simulink subsystem "Pid_Controller"  (R2025b)
settings: Solver=VariableStepAuto
undefined symbols (not defined in the file): bigBenUpright, pidGains
settings Model: Creator=ahmed medhat  LastModifiedBy=ahmed medhat

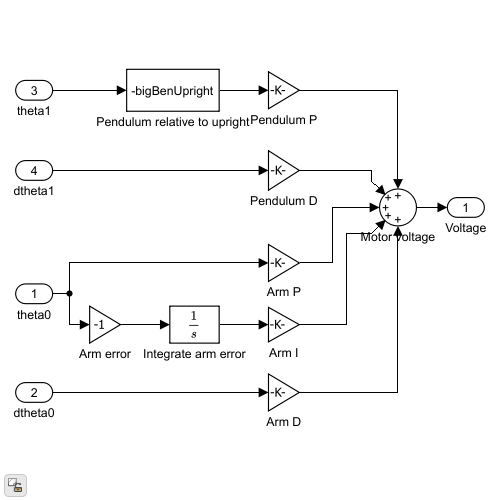
[thumbnail: Simulink's stored preview of the top-level diagram]
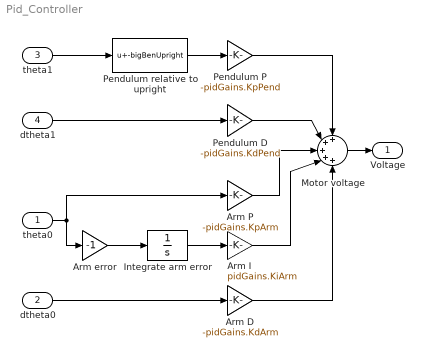
== system Pid_Controller ==
  theta0 : Inport
  dtheta0 : Inport  Port=2
  theta1 : Inport  Port=3
  dtheta1 : Inport  Port=4
  Arm D : Gain  Gain=-pidGains.KdArm
  Arm I : Gain  Gain=pidGains.KiArm
  Arm P : Gain  Gain=-pidGains.KpArm
  Arm error : Gain  Gain=-1
  Integrate arm error : Integrator
  Motor voltage : Sum  Inputs=+++++
  Pendulum D : Gain  Gain=-pidGains.KdPend
  Pendulum P : Gain  Gain=-pidGains.KpPend
  Pendulum relative to upright : Bias  Bias=-bigBenUpright  SaturateOnIntegerOverflow=off
  Voltage : Outport
  wires:
  theta0/1 -> Arm error/1, Arm P/1
  dtheta0/1 -> Arm D/1
  theta1/1 -> Pendulum relative to upright/1
  Pendulum relative to upright/1 -> Pendulum P/1
  dtheta1/1 -> Pendulum D/1
  Arm error/1 -> Integrate arm error/1
  Integrate arm error/1 -> Arm I/1
  Motor voltage/1 -> Voltage/1
  Arm D/1 -> Motor voltage/5
  Arm I/1 -> Motor voltage/4
  Arm P/1 -> Motor voltage/3
  Pendulum D/1 -> Motor voltage/2
  Pendulum P/1 -> Motor voltage/1
